simulink model "ElectricVehicleThermalManagementWithHeatPump"  (R2024b)
settings: Solver=VariableStepAuto  StartTime=0.0  StopTime=3600  RelTol=1e-3  AbsTol=1e-3
PreLoadFcn:
  | init_nmpc
InitFcn:
  | init_nmpc
model workspace: external: MATLAB File ElectricVehicleThermalManagementWithHeatPumpParameters.m (data not in the file)
values from neighbouring files (symbols this model uses):
  battery_C1_LUT = [1913.6 12447 30609 ... (first row only)    [ElectricVehicleThermalManagementWithHeatPumpParameters.m]
  battery_capacity_LUT = [280.081 276.25 276.392]    [ElectricVehicleThermalManagementWithHeatPumpParameters.m]
  battery_cell_cp = 795    [ElectricVehicleThermalManagementWithHeatPumpParameters.m]
  battery_cell_mass = 2.5    [ElectricVehicleThermalManagementWithHeatPumpParameters.m]
  battery_Em_LUT = [3.4966 3.5057 3.5148 ... (first row only)    [ElectricVehicleThermalManagementWithHeatPumpParameters.m]
  battery_N_cells = 20    [ElectricVehicleThermalManagementWithHeatPumpParameters.m]
  battery_Qe_init = 0    [ElectricVehicleThermalManagementWithHeatPumpParameters.m]
  battery_R0_LUT = [0.0117 0.0085 0.009 ... (first row only)    [ElectricVehicleThermalManagementWithHeatPumpParameters.m]
  battery_R1_LUT = [0.0109 0.0029 0.0013 ... (first row only)    [ElectricVehicleThermalManagementWithHeatPumpParameters.m]
  battery_SOC_LUT = [0; 0.1; 0.25; 0.5; 0.75; 0.9; 1]    [ElectricVehicleThermalManagementWithHeatPumpParameters.m]
  battery_T_init = -10    [ElectricVehicleThermalManagementWithHeatPumpParameters.m]
  battery_temperature_LUT = [5 20 40]    [ElectricVehicleThermalManagementWithHeatPumpParameters.m]
  cabin_duct_area = 0.04    [ElectricVehicleThermalManagementWithHeatPumpParameters.m]
  cabin_T_init = -10    [ElectricVehicleThermalManagementWithHeatPumpParameters.m]
  chiller_area_primary = 0.43982297150257105    (= 0.439822971503)    [ElectricVehicleThermalManagementWithHeatPumpParameters.m]
  chiller_N_baffles = 3    [ElectricVehicleThermalManagementWithHeatPumpParameters.m]
  chiller_N_tubes = 100    [ElectricVehicleThermalManagementWithHeatPumpParameters.m]
  chiller_tube_D = 0.0035    [ElectricVehicleThermalManagementWithHeatPumpParameters.m]
  chiller_tube_L = 0.4    [ElectricVehicleThermalManagementWithHeatPumpParameters.m]
  chiller_wall_conductivity = 240    [ElectricVehicleThermalManagementWithHeatPumpParameters.m]
  chiller_wall_thickness = 0.0001    [ElectricVehicleThermalManagementWithHeatPumpParameters.m]
  cond_evap_air_area_flow = 0.3906    [ElectricVehicleThermalManagementWithHeatPumpParameters.m]
  cond_evap_air_area_primary = 1.4834999999999998    (= 1.4835)    [ElectricVehicleThermalManagementWithHeatPumpParameters.m]
  cond_evap_W = 0.015    [ElectricVehicleThermalManagementWithHeatPumpParameters.m]
  cond_evap_wall_conductivity = 240    [ElectricVehicleThermalManagementWithHeatPumpParameters.m]
  cond_evap_wall_thickness = 0.0001    [ElectricVehicleThermalManagementWithHeatPumpParameters.m]
  coolant_channel_D = 0.0092    [ElectricVehicleThermalManagementWithHeatPumpParameters.m]
  coolant_pipe_D = 0.019    [ElectricVehicleThermalManagementWithHeatPumpParameters.m]
  coolant_T_init = -10    [ElectricVehicleThermalManagementWithHeatPumpParameters.m]
  coolant_tank_area = 0.0121    [ElectricVehicleThermalManagementWithHeatPumpParameters.m]
  coolant_tank_volume = 1.25    [ElectricVehicleThermalManagementWithHeatPumpParameters.m]
  coolant_valve_D_ratio_max = 0.95    [ElectricVehicleThermalManagementWithHeatPumpParameters.m]
  coolant_valve_D_ratio_min = 0.001    [ElectricVehicleThermalManagementWithHeatPumpParameters.m]
  coolant_valve_displacement = 0.0063    [ElectricVehicleThermalManagementWithHeatPumpParameters.m]
  coolant_valve_S_max = 0.0053    [ElectricVehicleThermalManagementWithHeatPumpParameters.m]
  evaporator_air_area_flow = 0.12    [ElectricVehicleThermalManagementWithHeatPumpParameters.m]
  evaporator_air_area_primary = 0.4323    [ElectricVehicleThermalManagementWithHeatPumpParameters.m]
  evaporator_W = 0.015    [ElectricVehicleThermalManagementWithHeatPumpParameters.m]
  evaporator_wall_conductivity = 240    [ElectricVehicleThermalManagementWithHeatPumpParameters.m]
  evaporator_wall_thickness = 0.0001    [ElectricVehicleThermalManagementWithHeatPumpParameters.m]
  expansion_valve_D_ratio_max = 0.9    [ElectricVehicleThermalManagementWithHeatPumpParameters.m]
  hex_area_primary = 0.070371675440411369    (= 0.0703716754404)    [ElectricVehicleThermalManagementWithHeatPumpParameters.m]
  hex_N_tubes = 64    [ElectricVehicleThermalManagementWithHeatPumpParameters.m]
  hex_tube_D = 0.0035    [ElectricVehicleThermalManagementWithHeatPumpParameters.m]
  hex_wall_conductivity = 240    [ElectricVehicleThermalManagementWithHeatPumpParameters.m]
  hex_wall_thickness = 0.0001    [ElectricVehicleThermalManagementWithHeatPumpParameters.m]
  inner_cond_air_area_flow = 0.1953    [ElectricVehicleThermalManagementWithHeatPumpParameters.m]
  inner_cond_air_area_primary = 0.99520000000000008    (= 0.9952)    [ElectricVehicleThermalManagementWithHeatPumpParameters.m]
  inner_cond_W = 0.02    [ElectricVehicleThermalManagementWithHeatPumpParameters.m]
  inner_cond_wall_conductivity = 240    [ElectricVehicleThermalManagementWithHeatPumpParameters.m]
  inner_cond_wall_thickness = 0.0001    [ElectricVehicleThermalManagementWithHeatPumpParameters.m]
  pump_speed_max = 1000    [ElectricVehicleThermalManagementWithHeatPumpParameters.m]
  radiator_air_area_flow = 0.097499999999999989    (= 0.0975)    [ElectricVehicleThermalManagementWithHeatPumpParameters.m]
  radiator_air_area_primary = 0.43687499999999996    (= 0.436875)    [ElectricVehicleThermalManagementWithHeatPumpParameters.m]
  radiator_W = 0.015    [ElectricVehicleThermalManagementWithHeatPumpParameters.m]
  radiator_wall_conductivity = 240    [ElectricVehicleThermalManagementWithHeatPumpParameters.m]
  radiator_wall_thickness = 0.0001    [ElectricVehicleThermalManagementWithHeatPumpParameters.m]
  refrigerant_p_init = 0.2    [ElectricVehicleThermalManagementWithHeatPumpParameters.m]
  refrigerant_pipe_D = 0.01    [ElectricVehicleThermalManagementWithHeatPumpParameters.m]
  refrigerant_valve_D_ratio_max = 0.95    [ElectricVehicleThermalManagementWithHeatPumpParameters.m]
  refrigerant_valve_displacement = 0.005    [ElectricVehicleThermalManagementWithHeatPumpParameters.m]
libraries: fl_lib x227, nesl_utility x162, SimscapeFluids_lib x30, LiBatteryElements_lib x16, slpidlib x3, SignalEditorBlockLib x1
(part 7 of 13)

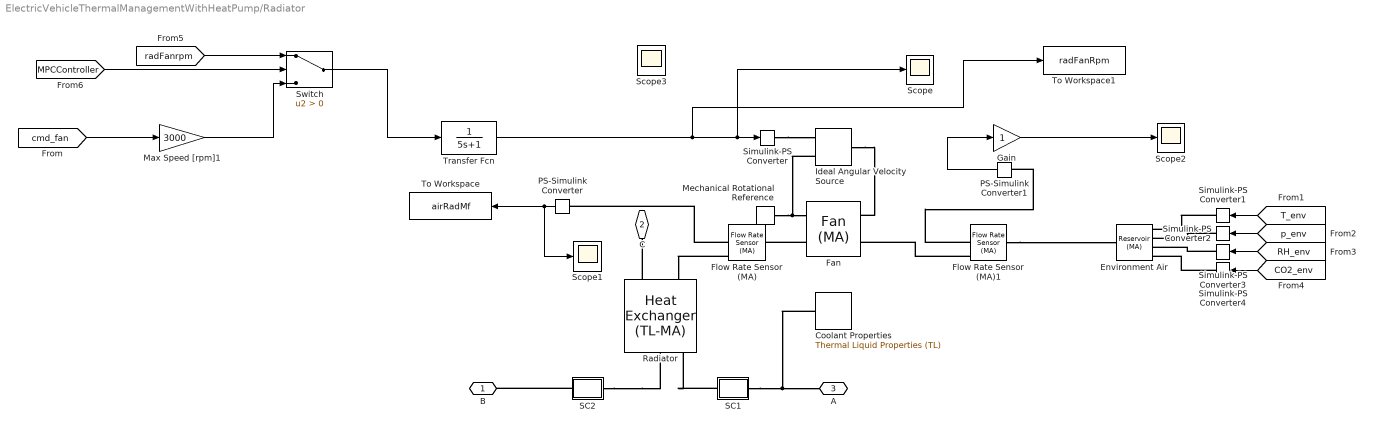
== system ElectricVehicleThermalManagementWithHeatPump/Radiator ==
  Coolant Properties : SimscapeFluids_lib/Thermal Liquid/Utilities/Thermal Liquid Properties (TL)  fluid_list=fluids.thermal_liquid.utilities.enum.thermal_liquid_fluid_list.ethylene_glycol  concentration_param_EG=fluids.thermal_liquid.utilities.enum.thermal_liquid_concentration.volume_fraction  concentration_param_PG=fluids.thermal_liquid.utilities.enum.thermal_liquid_concentration.volume_fraction  c_mass_SW=3.5e-3  c_mass_EG=0.1  c_mass_PG=0.1  c_mass_GL=0.1  c_vol_EG=0.5  c_vol_PG=0.1  beta_const_EG=2.1791 GPa  beta_const_PG=2.1791 GPa  beta_const_GL=2.1791 GPa  p_min_EG=0.01 MPa  p_min_PG=0.01 MPa  p_min_GL=0.01 MPa  p_max_EG=50 MPa  p_max_PG=50 MPa  p_max_GL=50 MPa  p_atm=0.101325 MPa  properties_range_check=simscape.enum.assert.action.error
  Environment Air : fl_lib/Moist Air/Elements/Reservoir (MA)  pressure_input=true  pressure_spec=foundation.enum.pressure_spec.atmospheric  reservoir_pressure=0.101325 MPa  temperature_input=true  temperature_spec=foundation.enum.temperature_spec.atmospheric  reservoir_temperature=293.15 K  humidity_input=true  humidity_spec=foundation.enum.HumiditySpec.RelativeHumidity  reservoir_RH=0.5  reservoir_x_w=0.01  reservoir_y_w=0.01  reservoir_HR=0.01  reservoir_Tw=287 K  trace_gas_input=true  trace_gas_spec=foundation.enum.trace_gas_spec.mole_fraction  reservoir_x_g=0.001  reservoir_y_g=0.001  water_droplets_input=false  reservoir_r_d=0  RH_ws=1  area_A=cabin_duct_area m^2  input_error_spec=foundation.enum.input_range_error.warn
      settings: InternalSimscapePortConfiguration="{\"Bottom\":[],\"Left\":[{\"id\":\"A\",\"label\":\"A\",\"type\":\"foundation.moist_air.moist_air\"}],\"Right\":[{\"id\":\"T\",\"label\":\"T\",\"type\":\"input\"},{\"id\":\"P\",\"label\":\"P\",\"type\":\"input\"},{\"id\":\"W\",\"label\":\"W\",\"type\":\"input\"},{\"id\":\"G\",\"label\":\"G\",\"type\":\"input\"}],\"Top\":[]}"
  Fan : SimscapeFluids_lib/Moist Air/Turbomachinery/Fan (MA)  fan_parameterization=fluids.moist_air.turbomachinery.enum.FanParameterization.Table1D  mechanical_power_spec=fluids.moist_air.turbomachinery.enum.FanMechanicalPowerSpec.Efficiency  flow_rate_nominal=0.8 m^3/s  pressure_nominal=400 Pa  eta_nominal=0.6  power_nominal=1620 W  pressure_max=600 Pa  flow_rate_max=1.5 m^3/s  omega_ref_nominal=1000 rpm  flow_rate_1D_TLU=[.0278, .0556, .0833, .111, .139, .167] m^3/s  pressure_1D_TLU=[6410, 6375, 6018, 5366, 4501, 3609] Pa  eta_1D_TLU=[.257, .394, .453, .47, .459, .415]  power_1D_TLU=[693, 900, 1107, 1267, 1363, 1452] W  omega_ref_1D=3000 rpm  rho_ref_1D=1.2 kg/m^3  omega_threshold_factor=1e-2  omega_dp_TLU=[2400; 3000; 3600] rpm  flow_rate_dp_TLU=[.0278, .0556, .0833, .111, .139, .167] m^3/s  pressure_dp_TLU=[4111, 4010, 3551, 2881, 2167, 1453; 6410, 6375, 6018, 5366, 4501, 3609; 9217, 9285, 9022, 8428, 7552, 6482] Pa  eta_dp_TLU=[.3, .434, .468, .459, .4, .3; .257, .394, .453, .47, .459, .415; .225, .359, .434, .461, .47, .459]  power_dp_TLU=[381, 514, 632, 697, 753, 809; 693, 900, 1107, 1267, 1363, 1452; 1139, 1438, 1732, 2029, 2233, 2358] W  rho_ref_dp=1.2 kg/m^3  omega_q_TLU=[2990; 3450; 3867] rpm  pressure_q_TLU=[31, 62, 93, 124] Pa  flow_rate_q_TLU=[.802, .759, .703, .611; .936, .902, .862, .81; 1.056, 1.027, .994, .956] m^3/s  eta_q_TLU=[.088, .162, .22, .261; .068, .128, .18, .222; .055, .105, .148, .188]  power_q_TLU=[283, 290, 297, 290; 427, 437, 445, 452; 595, 606, 625, 631] W  rho_ref_q=1.2 kg/m^3  diameter_ratio=1  mech_orientation=fluids.moist_air.turbomachinery.enum.FanMechanicalOrientation.Positive  area_A=cabin_duct_area m^2  area_B=cabin_duct_area m^2
      settings: InternalSimscapePortConfiguration="{\"Bottom\":[],\"Left\":[{\"id\":\"A\",\"label\":\"A\",\"type\":\"foundation.moist_air.moist_air\"},{\"id\":\"C\",\"label\":\"C\",\"type\":\"foundation.mechanical.rotational.rotational\"}],\"Right\":[{\"id\":\"B\",\"label\":\"B\",\"type\":\"foundation.moist_air.moist_air\"},{\"id\":\"R\",\"label\":\"R\",\"type\":\"foundation.mechanical.rotational.rotational\"}],\"Top\":[]}"
  Flow Rate Sensor (MA) : fl_lib/Moist Air/Sensors/Flow Rate Sensor (MA)  mass_flow_measure=true  volumetric_flow_measure=false  volumetric_flow_conditions=foundation.enum.volumetric_flow_conditions.actual  p_std=0.101325 MPa  T_std=20 degC  RH_std=0.65  energy_flow_measure=true  vapor_flow_measure=false  gas_flow_measure=false  droplets_flow_measure=false
      settings: InternalSimscapePortConfiguration="{\"Bottom\":[{\"id\":\"PHI\",\"label\":\"φ\",\"type\":\"output\"}],\"Left\":[{\"id\":\"A\",\"label\":\"A\",\"type\":\"foundation.moist_air.moist_air\"}],\"Right\":[{\"id\":\"B\",\"label\":\"B\",\"type\":\"foundation.moist_air.moist_air\"},{\"id\":\"M\",\"label\":\"M\",\"type\":\"output\"}],\"Top\":[]}"
  Flow Rate Sensor (MA)1 : fl_lib/Moist Air/Sensors/Flow Rate Sensor (MA)  mass_flow_measure=true  volumetric_flow_measure=false  volumetric_flow_conditions=foundation.enum.volumetric_flow_conditions.actual  p_std=0.101325 MPa  T_std=20 degC  RH_std=0.65  energy_flow_measure=true  vapor_flow_measure=false  gas_flow_measure=false  droplets_flow_measure=false
      settings: InternalSimscapePortConfiguration="{\"Bottom\":[{\"id\":\"PHI\",\"label\":\"φ\",\"type\":\"output\"}],\"Left\":[{\"id\":\"A\",\"label\":\"A\",\"type\":\"foundation.moist_air.moist_air\"}],\"Right\":[{\"id\":\"B\",\"label\":\"B\",\"type\":\"foundation.moist_air.moist_air\"},{\"id\":\"M\",\"label\":\"M\",\"type\":\"output\"}],\"Top\":[]}"
  Gain : Gain
  Ideal Angular Velocity Source : fl_lib/Mechanical/Mechanical Sources/Ideal Angular Velocity Source
  Max Speed [rpm]1 : Gain  Gain=3000
  Mechanical Rotational Reference : fl_lib/Mechanical/Rotational Elements/Mechanical Rotational Reference
  PS-Simulink Converter : nesl_utility/PS-Simulink Converter  PhysicalDomain=network_engine_domain  SubClassName=ps_output  LeftPortType=input  RightPortType=output  PseudoPeriodic=off  Frequencies=[]  VectorFormat=inherit  Unit=inherit  AffineConversion=off
  PS-Simulink Converter1 : nesl_utility/PS-Simulink Converter  PhysicalDomain=network_engine_domain  SubClassName=ps_output  LeftPortType=input  RightPortType=output  PseudoPeriodic=off  Frequencies=[]  VectorFormat=inherit  Unit=inherit  AffineConversion=off
  Radiator : SimscapeFluids_lib/Heat Exchangers/Thermal Liquid - Moist Air/Heat Exchanger (TL-MA)  flow_arrangement=fluids.heat_exchangers.enum.FlowArrangementTLMA.Cross  cross_flow_arrangement=fluids.heat_exchangers.enum.CrossFlowArrangementTLMA.MixedUnmixed  R_wall=radiator_wall_thickness / radiator_air_area_primary / radiator_wall_conductivity K/W  area_A1=pi * coolant_pipe_D^2 / 4 m^2  area_B1=pi * coolant_pipe_D^2 / 4 m^2  area_A2=cabin_duct_area m^2  area_B2=cabin_duct_area m^2  flow_geometry_TL=fluids.heat_exchangers.enum.FlowGeometryTL.InsideTubes  tube_num_TL=radiator_N_tubes  tube_length_TL=radiator_L m  tube_cross_section_TL=fluids.heat_exchangers.enum.TubeCrossSection.Rectangular  tube_diameter_TL=0.1 m  tube_width_TL=radiator_W m  tube_height_TL=radiator_tube_H m  tube_inner_diameter_TL=0.05 m  tube_outer_diameter_TL=0.1 m  tube_flow_area_TL=0.01 m^2  tube_wetted_perimeter_TL=0.4 m  tube_heat_perimeter_TL=0.4 m  tube_pressure_loss_spec_TL=fluids.heat_exchangers.enum.TubePressureLossSpec.Haaland  tube_loss_coeff_TL=10  tube_local_pressure_loss_spec_TL=fluids.heat_exchangers.enum.LocalLossSpec.AggregateLength  tube_length_add_TL=radiator_tube_Leq m  tube_local_loss_coefficient_TL=0.1  tube_roughness_pressure_TL=15e-6 m  tube_Re_lam_pressure_TL=2000  tube_Re_tur_pressure_TL=4000  tube_shape_factor_generic_TL=64  tube_heat_coeff_spec_TL=fluids.heat_exchangers.enum.TubeHeatCoeffSpec.Gneilinski  tube_colburn_coeff_TL=[.023, .8, .33]  tube_roughness_heat_TL=15e-6 m  tube_Re_lam_heat_TL=2000  tube_Re_tur_heat_TL=4000  tube_Nu_lam_generic_TL=3.66  bank_arrangement_TL=fluids.heat_exchangers.enum.BankArrangement.Inline  bank_num_rows_TL=5  bank_tubes_per_row_TL=5  bank_width_TL=1 m  bank_tube_diameter_TL=0.05 m  bank_longitudinal_pitch_TL=0.15 m  bank_transverse_pitch_TL=0.15 m  bank_pressure_loss_spec_TL=fluids.heat_exchangers.enum.BankPressureLossSpec.Martin  bank_euler_TL=10  bank_heat_coeff_spec_TL=fluids.heat_exchangers.enum.BankHeatCoeffSpec.Martin  bank_colburn_coeff_TL=[.27, .63, .36]  generic_flow_area_TL=0.01 m^2  generic_heat_area_TL=2 m^2  generic_volume_TL=0.05 m^3  generic_loss_coeff_TL=10  generic_colburn_coeff_TL=[.023, .8, .33]  fouling_factor_TL=0.1 m^2*K/kW  fin_area_TL=0 m^2  fin_efficiency_TL=0  p_init_TL=coolant_p_init MPa  T_init_TL=coolant_T_init degC  flow_geometry_MA=fluids.heat_exchangers.enum.FlowGeometryMA.Generic  tube_num_MA=1  tube_length_MA=5 m  tube_cross_section_MA=fluids.heat_exchangers.enum.TubeCrossSection.Circular  tube_diameter_MA=0.1 m  tube_width_MA=0.1 m  tube_height_MA=0.1 m  tube_inner_diameter_MA=0.05 m  tube_outer_diameter_MA=0.1 m  tube_flow_area_MA=0.01 m^2  tube_wetted_perimeter_MA=0.4 m  tube_heat_perimeter_MA=0.4 m  tube_pressure_loss_spec_MA=fluids.heat_exchangers.enum.TubePressureLossSpec.Haaland  tube_loss_coeff_MA=10  tube_local_pressure_loss_spec_MA=fluids.heat_exchangers.enum.LocalLossSpec.AggregateLength  tube_length_add_MA=0.1 m  tube_local_loss_coefficient_MA=0.1  tube_roughness_pressure_MA=15e-6 m  tube_Re_lam_pressure_MA=2000  tube_Re_tur_pressure_MA=4000  tube_shape_factor_generic_MA=64  tube_heat_coeff_spec_MA=fluids.heat_exchangers.enum.TubeHeatCoeffSpec.Gneilinski  tube_colburn_coeff_MA=[.023, .8, .33]  tube_roughness_heat_MA=15e-6 m  tube_Re_lam_heat_MA=2000  tube_Re_tur_heat_MA=4000  tube_Nu_lam_generic_MA=3.66  bank_arrangement_MA=fluids.heat_exchangers.enum.BankArrangement.Inline  bank_num_rows_MA=5  bank_tubes_per_row_MA=5  bank_width_MA=1 m  bank_tube_diameter_MA=0.05 m  bank_longitudinal_pitch_MA=0.15 m  bank_transverse_pitch_MA=0.15 m  bank_pressure_loss_spec_MA=fluids.heat_exchangers.enum.BankPressureLossSpec.Martin  bank_euler_MA=10  bank_heat_coeff_spec_MA=fluids.heat_exchangers.enum.BankHeatCoeffSpec.Martin  bank_colburn_coeff_MA=[.27, .63, .36]  generic_flow_area_MA=radiator_air_area_flow m^2  generic_heat_area_MA=radiator_air_area_primary m^2  generic_volume_MA=radiator_air_area_flow * radiator_W m^3  generic_loss_coeff_MA=10  generic_colburn_coeff_MA=[0.27, 0.63, 0.36]  fouling_factor_MA=0.1 m^2*K/kW  fin_area_MA=radiator_air_area_fins m^2  fin_efficiency_MA=0.7  p_init_MA=cabin_p_init MPa  T_init_MA=cabin_T_init degC  humidity_spec_MA=foundation.enum.HumiditySpec.RelativeHumidity  RH_init_MA=cabin_RH_init  x_w_init_MA=0.01  y_w_init_MA=0.01  HR_init_MA=0.01  Tw_init_MA=287 K  trace_gas_spec_MA=foundation.enum.trace_gas_spec.mole_fraction  x_g_init_MA=0.001  y_g_init_MA=cabin_CO2_init  r_d_init_MA=0  RH_ws_MA=1  time_constant_cond_MA=1e-3 s  time_constant_evap_MA=1e-3 s  fraction_entrained_MA=1
      settings: InternalSimscapePortConfiguration="{\"Bottom\":[],\"Left\":[{\"id\":\"A1\",\"label\":\"A1\",\"type\":\"foundation.thermal_liquid.thermal_liquid\"},{\"id\":\"B1\",\"label\":\"B1\",\"type\":\"foundation.thermal_liquid.thermal_liquid\"}],\"Right\":[{\"id\":\"A2\",\"label\":\"A2\",\"type\":\"foundation.moist_air.moist_air\"},{\"id\":\"B2\",\"label\":\"B2\",\"type\":\"foundation.moist_air.moist_air\"}],\"Top\":[{\"id\":\"W\",\"label\":\"W\",\"type\":\"output\"}]}"
  SC1 : Subsystem
  SC2 : Subsystem
  Scope{,1..3} (4 alike) : Scope
  Simulink-PS Converter : nesl_utility/Simulink-PS Converter  PhysicalDomain=network_engine_domain  SubClassName=ps_input  LeftPortType=input  RightPortType=output  PseudoPeriodic=off  Frequencies=[]  NoiseDistribution=none  NoiseParameters=[]  Unit=rpm  AffineConversion=off  FilteringAndDerivatives=provide  SimscapeFilterOrder=1  InputFilterTimeConstant=0.001  UdotUserProvided=0
  Simulink-PS Converter1 : nesl_utility/Simulink-PS Converter  PhysicalDomain=network_engine_domain  SubClassName=ps_input  LeftPortType=input  RightPortType=output  PseudoPeriodic=off  Frequencies=[]  NoiseDistribution=none  NoiseParameters=[]  Unit=degC  AffineConversion=on  FilteringAndDerivatives=provide  SimscapeFilterOrder=1  InputFilterTimeConstant=0.001  UdotUserProvided=0
  Simulink-PS Converter2 : nesl_utility/Simulink-PS Converter  PhysicalDomain=network_engine_domain  SubClassName=ps_input  LeftPortType=input  RightPortType=output  PseudoPeriodic=off  Frequencies=[]  NoiseDistribution=none  NoiseParameters=[]  Unit=MPa  AffineConversion=off  FilteringAndDerivatives=provide  SimscapeFilterOrder=1  InputFilterTimeConstant=0.001  UdotUserProvided=0
  Simulink-PS Converter3 : nesl_utility/Simulink-PS Converter  PhysicalDomain=network_engine_domain  SubClassName=ps_input  LeftPortType=input  RightPortType=output  PseudoPeriodic=off  Frequencies=[]  NoiseDistribution=none  NoiseParameters=[]  Unit=1  AffineConversion=off  FilteringAndDerivatives=provide  SimscapeFilterOrder=1  InputFilterTimeConstant=0.001  UdotUserProvided=0
  Simulink-PS Converter4 : nesl_utility/Simulink-PS Converter  PhysicalDomain=network_engine_domain  SubClassName=ps_input  LeftPortType=input  RightPortType=output  PseudoPeriodic=off  Frequencies=[]  NoiseDistribution=none  NoiseParameters=[]  Unit=1  AffineConversion=off  FilteringAndDerivatives=provide  SimscapeFilterOrder=1  InputFilterTimeConstant=0.001  UdotUserProvided=0
  Switch : Switch  Criteria=u2 > Threshold  SaturateOnIntegerOverflow=off  InputSameDT=off
  To Workspace : ToWorkspace  VariableName=airRadMf  SampleTime=-1
  To Workspace1 : ToWorkspace  VariableName=radFanRpm  SampleTime=-1
  Transfer Fcn : TransferFcn  Denominator=[5 1]
  B : PMIOPort  Side=Left
  C : PMIOPort  Port=2  Side=Left
  A : PMIOPort  Port=3  Side=Right
  wires:
  [T_env] -> Simulink-PS Converter1/1
  [p_env] -> Simulink-PS Converter2/1
  [RH_env] -> Simulink-PS Converter3/1
  [CO2_env] -> Simulink-PS Converter4/1
  PS-Simulink Converter/1 -> Scope1/1, To Workspace/1
  PS-Simulink Converter1/1 -> Gain/1
  Gain/1 -> Scope2/1
  Transfer Fcn/1 -> To Workspace1/1, Scope/1, Simulink-PS Converter/1
  [radFanrpm] -> Switch/1
  [cmd_fan] -> Max Speed [rpm]1/1
  Switch/1 -> Transfer Fcn/1
  Max Speed [rpm]1/1 -> Switch/3
  [MPCController] -> Switch/2
  connections:
  SC2/LConn1 -- Radiator/LConn2
  SC1/RConn1 -- Radiator/LConn1
  Radiator/RConn2 -- C/RConn1
  Simulink-PS Converter2/RConn1 -- Environment Air/RConn2
  Simulink-PS Converter4/RConn1 -- Environment Air/RConn4
  Simulink-PS Converter3/RConn1 -- Environment Air/RConn3
  Simulink-PS Converter1/RConn1 -- Environment Air/RConn1
  SC2/RConn1 -- B/RConn1
  SC1/LConn1 -- Coolant Properties/RConn1 -- A/RConn1
  Ideal Angular Velocity Source/RConn2 -- Mechanical Rotational Reference/LConn1 -- Fan/LConn2
  Simulink-PS Converter/RConn1 -- Ideal Angular Velocity Source/RConn1
  Ideal Angular Velocity Source/LConn1 -- Fan/RConn2
  Fan/LConn1 -- Flow Rate Sensor (MA)/LConn1
  Flow Rate Sensor (MA)/RConn1 -- Radiator/RConn1
  Flow Rate Sensor (MA)/RConn2 -- PS-Simulink Converter/LConn1
  Flow Rate Sensor (MA)1/LConn1 -- Environment Air/LConn1
  Flow Rate Sensor (MA)1/RConn1 -- Fan/RConn1
  Flow Rate Sensor (MA)1/RConn2 -- PS-Simulink Converter1/LConn1

== system ElectricVehicleThermalManagementWithHeatPump/Radiator Bypass Valve ==
  Bias : Bias  Bias=-1  SaturateOnIntegerOverflow=off
  Gain : Gain  Gain=2
  Max Valve Displacement [m] : Gain  Gain=coolant_valve_displacement
  Radiator Bypass Valve : SimscapeFluids_lib/Thermal Liquid/Valves & Orifices/Directional Control Valves/3-Way Directional Valve (TL)  open_orifices_pos=fluids.thermal_liquid.valves.directional_control_valves.enum.OpenOrifices3Way.PA  open_orifices_neg=fluids.thermal_liquid.valves.directional_control_valves.enum.OpenOrifices3Way.AT  area_spec=fluids.thermal_liquid.valves.directional_control_valves.enum.area_spec.identical  valve_spec=fluids.thermal_liquid.valves.enum.orifice_spec.linear  del_S_max=coolant_valve_displacement m  area_max=pi * (coolant_valve_D_ratio_max*coolant_pipe_D)^2 / 4 m^2  del_S_TLU=[0 0.002 0.004 0.007 0.017] m  valve_area_TLU=[1e-09, 2.0352e-07, 4.0736e-05, .00011438, .00034356] m^2  del_S_flow_TLU=[0 0.002 0.004 0.007 0.017] m  p_diff_TLU=[-.1, .3, .5, .7] MPa  vol_flow_TLU=1e-3 * [1.7e-05, 2e-05, 2.6e-05; .0035, .0045, .0053; .7, .9, 1.06; 1.96, 2.5, 3; 6, 7.7, 9.13] m^3/s  mdot_TLU=[-1e-05, 1.7e-05, 2e-05, 2.6e-05; -.002, .0035, .0045, .0053; -.4, .7, .9, 1.06; -1.13, 1.96, 2.5, 3; -3.45, 6, 7.7, 9.13] kg/s  T_ref_in=293.15 K  p_ref_in=0.101325 MPa  area_leak=pi * (coolant_valve_D_ratio_min*coolant_pipe_D)^2 / 4 m^2  Cd=0.7  Re_c=150  smoothing_factor=0.01  pressure_recovery=simscape.enum.onoff.on  area=pi * coolant_pipe_D^2 / 4 m^2  S_max_PA=coolant_valve_S_max m  del_S_max_PA=coolant_valve_displacement-(coolant_valve_displacement)*(pi * (coolant_valve_D_ratio_min*coolant_pipe_D)^2 / 4)/(pi * (coolant_valve_D_ratio_max*coolant_pipe_D)^2 / 4) m  area_max_PA=pi * (coolant_valve_D_ratio_max*coolant_pipe_D)^2 / 4 m^2  del_S_TLU_PA=[0 0.002 0.004 0.007 0.017] m  valve_area_TLU_PA=[1e-09, 2.0352e-07, 4.0736e-05, .00011438, .00034356] m^2  del_S_flow_TLU_PA=[0 0.002 0.004 0.007 0.017] m  p_diff_TLU_PA=[-.1, .3, .5, .7] MPa  vol_flow_TLU_PA=1e-3 * [1.7e-05, 2e-05, 2.6e-05; .0035, .0045, .0053; .7, .9, 1.06; 1.96, 2.5, 3; 6, 7.7, 9.13] m^3/s  mdot_TLU_PA=[-1e-05, 1.7e-05, 2e-05, 2.6e-05; -.002, .0035, .0045, .0053; -.4, .7, .9, 1.06; -1.13, 1.96, 2.5, 3; -3.45, 6, 7.7, 9.13] kg/s  S_max_AT=-coolant_valve_S_max m  del_S_max_AT=coolant_valve_displacement-(coolant_valve_displacement)*(pi * (coolant_valve_D_ratio_min*coolant_pipe_D)^2 / 4)/(pi * (coolant_valve_D_ratio_max*coolant_pipe_D)^2 / 4) m  area_max_AT=pi * (coolant_valve_D_ratio_max*coolant_pipe_D)^2 / 4 m^2  del_S_TLU_AT=[0 0.002 0.004 0.007 0.017] m  valve_area_TLU_AT=[1e-09, 2.0352e-07, 4.0736e-05, .00011438, .00034356] m^2  del_S_flow_TLU_AT=[0 0.002 0.004 0.007 0.017] m  p_diff_TLU_AT=[-.1, .3, .5, .7] MPa  vol_flow_TLU_AT=1e-3 * [1.7e-05, 2e-05, 2.6e-05; .0035, .0045, .0053; .7, .9, 1.06; 1.96, 2.5, 3; 6, 7.7, 9.13] m^3/s  mdot_TLU_AT=[-1e-05, 1.7e-05, 2e-05, 2.6e-05; -.002, .0035, .0045, .0053; -.4, .7, .9, 1.06; -1.13, 1.96, 2.5, 3; -3.45, 6, 7.7, 9.13] kg/s  S_max_PT=2.5e-3 m  del_S_max_PT=0.005 m  area_max_PT=1e-4 m^2  del_S_TLU_PT=[0, .002, .004, .007, .017] m  valve_area_TLU_PT=[1e-09, 2.0352e-07, 4.0736e-05, .00011438, .00034356] m^2  del_S_flow_TLU_PT=[0, .002, .004, .007, .017] m  p_diff_TLU_PT=[.3, .5, .7] MPa  vol_flow_TLU_PT=1e-3 * [1.7e-05, 2e-05, 2.6e-05; .0035, .0045, .0053; .7, .9, 1.06; 1.96, 2.5, 3; 6, 7.7, 9.13] m^3/s  mdot_TLU_PT=[1.7e-05, 2e-05, 2.6e-05; .0035, .0045, .0053; .7, .9, 1.06; 1.96, 2.5, 3; 6, 7.7, 9.13] kg/s
      settings: InternalSimscapePortConfiguration="{\"Bottom\":[],\"Left\":[{\"id\":\"A\",\"label\":\"A\",\"type\":\"foundation.thermal_liquid.thermal_liquid\"}],\"Right\":[{\"id\":\"S\",\"label\":\"S\",\"type\":\"input\"},{\"id\":\"P\",\"label\":\"P\",\"type\":\"foundation.thermal_liquid.thermal_liquid\"},{\"id\":\"T\",\"label\":\"T\",\"type\":\"foundation.thermal_liquid.thermal_liquid\"}],\"Top\":[]}"
  Scope : Scope
  Simulink-PS Converter : nesl_utility/Simulink-PS Converter  PhysicalDomain=network_engine_domain  SubClassName=ps_input  LeftPortType=input  RightPortType=output  PseudoPeriodic=off  Frequencies=[]  NoiseDistribution=none  NoiseParameters=[]  Unit=m  AffineConversion=off  FilteringAndDerivatives=provide  SimscapeFilterOrder=1  InputFilterTimeConstant=0.001  UdotUserProvided=0
  Transfer Fcn : TransferFcn  Denominator=[1 1]
  B : PMIOPort  Side=Left
  C : PMIOPort  Port=2  Side=Left
  A : PMIOPort  Port=3  Side=Right
  wires:
  Gain/1 -> Bias/1
  [cmd_rad_bypass] -> Scope/1, Transfer Fcn/1
  Bias/1 -> Max Valve Displacement [m]/1
  Transfer Fcn/1 -> Gain/1
  Max Valve Displacement [m]/1 -> Simulink-PS Converter/1
  connections:
  Radiator Bypass Valve/LConn1 -- A/RConn1
  B/RConn1 -- Radiator Bypass Valve/RConn2
  Radiator Bypass Valve/RConn1 -- Simulink-PS Converter/RConn1
  Radiator Bypass Valve/RConn3 -- C/RConn1

== system ElectricVehicleThermalManagementWithHeatPump/Scenario ==
  note: Environment
  note: Cabin HVAC
  CO2 Fraction : Constant  Value=4e-4
  Clock : Clock
  Desired Temperature [degC] : Constant  Value=21
  Number of Occupants : Constant
  Power Demand : Subsystem
  Pressure [MPa] : Constant  Value=0.101325
  Relative Humidity : Constant  Value=0.5
  Scope : Scope
  Scope1 : Scope
  Scope2 : Scope
  Temperature [degC] : Constant  Value=-10
  Temperature [degC] vs Time : Lookup_n-D  NumberOfTableDimensions=1  BreakpointsForDimension1=[0 1150 1800 3600]  Table=[25 25 5 5]  InternalRulePriority=Speed  RndMeth=Simplest
  To Workspace : ToWorkspace  VariableName=batA_meas  SampleTime=-1
  Variant Source : VariantSource  VariantControlMode=label  LabelModeActiveChoice=constant
      settings: AttributesFormatString=%<LabelModeActiveChoice>
  Vehicle Speed [km/hr] : SignalEditorBlockLib/Signal Editor  FileName=ElectricVehicleThermalManagementWithHeatPumpVehicleSpeed.mat  ActiveScenario=DriveCycle  ActiveSignal=speed  IsBus=off  OutputBusObjectStr=Bus: BusObject  SampleTime=0  ZeroCross=off  OutputAfterFinalValue=Extrapolation  Unit=inherit  PreserveSignalName=on  ApplySigPropsToAllScenarios=on  ApplySigPropsToAllSignals=off
  tag scope: CO2_env=global, I_battery=global, N_occupant=global, Q_charger=global, Q_dcdc=global, Q_inverter=global, Q_motor=global, RH_env=global, T_desired=global, T_env=global, p_env=global, v_vehicle=global
  wires:
  Vehicle Speed [km/hr]/1 -> [v_vehicle], Power Demand/1(speed)
  Pressure [MPa]/1 -> [p_env]
  CO2 Fraction/1 -> [CO2_env]
  Desired Temperature [degC]/1 -> [T_desired]
  Relative Humidity/1 -> [RH_env]
  Power Demand/1(I_battery) -> To Workspace/1, Scope1/1, [I_battery]
  Power Demand/2(Q_inverter) -> [Q_inverter]
  Power Demand/3(Q_motor) -> Scope2/1, [Q_motor]
  Power Demand/4(Q_charger) -> [Q_charger]
  Power Demand/5(Q_dcdc) -> Scope/1, [Q_dcdc]
  Number of Occupants/1 -> [N_occupant]
  Variant Source/1 -> [T_env]
  Temperature [degC]/1 -> Variant Source/1
  Clock/1 -> Temperature [degC] vs Time/1
  Temperature [degC] vs Time/1 -> Variant Source/2

== system ElectricVehicleThermalManagementWithHeatPump/Battery/Pack 1 ==
  note: Scale up voltage drop
      | to total of N cells
  Controlled Voltage Source : fl_lib/Electrical/Electrical Sources/Controlled Voltage Source
  Lithium Cell 1RC : Subsystem
      settings: PortSchema="{\"entries\":[{\"content\":{\"sides\":[{\"content\":{\"connectorIds\":[]},\"type\":\"ConnectorPlacement.EquallySpacedRectSide\",\"uuid\":\"ccb9f794-c2a7-49a2-9836-26607ca18a9f\"},{\"content\":{\"connectorIds\":[],\"side\":\"RIGHT\"},\"type\":\"ConnectorPlacement.EquallySpacedRectSide\",\"uuid\":\"f1620ab9-2b03-42d4-871e-d35b8093f316\"},{\"content\":{\"connectorIds\":[\"LConn1\",\"LConn2\"],\"side\":\"TOP\"},\"type\":\"ConnectorPlacement.EquallySpacedRectSide\",\"uuid\":\"e679b0d8-ccbe-4539-8d6b-f3ffcd05b92b\"},{\"content\":{\"connectorIds\":[\"RConn1\",\"RConn2\"],\"side\":\"BOTTOM\"},\"type\":\"ConnectorPlacement.EquallySpacedRectSide\",\"uuid\":\"2833ed9d-c0e8-49c1-ad7b-8d4bc87d1df9\"},{\"content\":{\"connectorIds\":[],\"side\":\"HIDDEN\"},\"type\":\"ConnectorPlacement.EquallySpacedRectSide\",\"uuid\":\"76338804-e613-4140-a6be-ae9642a12407\"}]},\"type\":\"ConnectorPlacement.EquallySpacedConnector\",\"uuid\":\"276130fc-4c62-4f99-ae12-f3121ff878f4\"}],\"packageUris\":[\"http://schema.mathworks.com/mf0/Connector/R2020b\"],\"version\":\"1.0\"}"
      mask Display:
      | % Battery icon
      | plot([0 0 0.8 0.8], [0.2 0.9 0.9 1.5])
      | plot([0 0 0.8 0.8], -[0.2 0.9 0.9 1.5])
      | patch([-0.4 0.4 0.4 -0.4], [-0.45 -0.45 -0.15 -0.15], [0 0 0])
      | patch([-0.9 0.9 0.9 -0.9], [0.15 0.15 0.45 0.45], [0 0 0])
      | 
      | % Plot points to set plot range
      | color('white')
      | plot(1.5,1.5)
      | plot(-1.5,-1.5)
      | 
      | % Port labels
      | color('red')
      | port_label('LConn',1,'P')
      | port_label('LConn',2,'+')
      | port_label('RConn',1,'T')
      | port_label('RConn',2,'-')
  N : fl_lib/Physical Signals/Functions/PS Gain  gain=Ncells
  N-1 : fl_lib/Physical Signals/Functions/PS Gain  gain=Ncells - 1
  Thermal Model : Subsystem
  Voltage Sensor : fl_lib/Electrical/Electrical Sensors/Voltage Sensor
  - : PMIOPort  Side=Right
  H : PMIOPort  Port=2  Side=Left
  + : PMIOPort  Port=3  Side=Left
  connections:
  N/RConn1 -- Thermal Model/LConn2
  H/RConn1 -- Thermal Model/LConn1
  -/RConn1 -- Controlled Voltage Source/RConn2
  N-1/RConn1 -- Controlled Voltage Source/RConn1
  +/RConn1 -- Lithium Cell 1RC/LConn2 -- Voltage Sensor/LConn1
  Voltage Sensor/RConn1 -- N-1/LConn1
  Lithium Cell 1RC/RConn2 -- Voltage Sensor/RConn2 -- Controlled Voltage Source/LConn1
  Lithium Cell 1RC/RConn1 -- Thermal Model/RConn1
  Lithium Cell 1RC/LConn1 -- N/LConn1

== system ElectricVehicleThermalManagementWithHeatPump/Battery/Pack 2 ==
  note: Scale up voltage drop
      | to total of N cells
  Controlled Voltage Source : fl_lib/Electrical/Electrical Sources/Controlled Voltage Source
  Lithium Cell 1RC : Subsystem
      settings: PortSchema="{\"entries\":[{\"content\":{\"sides\":[{\"content\":{\"connectorIds\":[]},\"type\":\"ConnectorPlacement.EquallySpacedRectSide\",\"uuid\":\"ccb9f794-c2a7-49a2-9836-26607ca18a9f\"},{\"content\":{\"connectorIds\":[],\"side\":\"RIGHT\"},\"type\":\"ConnectorPlacement.EquallySpacedRectSide\",\"uuid\":\"f1620ab9-2b03-42d4-871e-d35b8093f316\"},{\"content\":{\"connectorIds\":[\"LConn1\",\"LConn2\"],\"side\":\"TOP\"},\"type\":\"ConnectorPlacement.EquallySpacedRectSide\",\"uuid\":\"e679b0d8-ccbe-4539-8d6b-f3ffcd05b92b\"},{\"content\":{\"connectorIds\":[\"RConn1\",\"RConn2\"],\"side\":\"BOTTOM\"},\"type\":\"ConnectorPlacement.EquallySpacedRectSide\",\"uuid\":\"2833ed9d-c0e8-49c1-ad7b-8d4bc87d1df9\"},{\"content\":{\"connectorIds\":[],\"side\":\"HIDDEN\"},\"type\":\"ConnectorPlacement.EquallySpacedRectSide\",\"uuid\":\"76338804-e613-4140-a6be-ae9642a12407\"}]},\"type\":\"ConnectorPlacement.EquallySpacedConnector\",\"uuid\":\"276130fc-4c62-4f99-ae12-f3121ff878f4\"}],\"packageUris\":[\"http://schema.mathworks.com/mf0/Connector/R2020b\"],\"version\":\"1.0\"}"
      mask Display:
      | % Battery icon
      | plot([0 0 0.8 0.8], [0.2 0.9 0.9 1.5])
      | plot([0 0 0.8 0.8], -[0.2 0.9 0.9 1.5])
      | patch([-0.4 0.4 0.4 -0.4], [-0.45 -0.45 -0.15 -0.15], [0 0 0])
      | patch([-0.9 0.9 0.9 -0.9], [0.15 0.15 0.45 0.45], [0 0 0])
      | 
      | % Plot points to set plot range
      | color('white')
      | plot(1.5,1.5)
      | plot(-1.5,-1.5)
      | 
      | % Port labels
      | color('red')
      | port_label('LConn',1,'P')
      | port_label('LConn',2,'+')
      | port_label('RConn',1,'T')
      | port_label('RConn',2,'-')
  N : fl_lib/Physical Signals/Functions/PS Gain  gain=Ncells
  N-1 : fl_lib/Physical Signals/Functions/PS Gain  gain=Ncells - 1
  Thermal Model : Subsystem
  Voltage Sensor : fl_lib/Electrical/Electrical Sensors/Voltage Sensor
  - : PMIOPort  Side=Right
  H : PMIOPort  Port=2  Side=Left
  + : PMIOPort  Port=3  Side=Left
  connections:
  N/RConn1 -- Thermal Model/LConn2
  H/RConn1 -- Thermal Model/LConn1
  -/RConn1 -- Controlled Voltage Source/RConn2
  N-1/RConn1 -- Controlled Voltage Source/RConn1
  +/RConn1 -- Lithium Cell 1RC/LConn2 -- Voltage Sensor/LConn1
  Voltage Sensor/RConn1 -- N-1/LConn1
  Lithium Cell 1RC/RConn2 -- Voltage Sensor/RConn2 -- Controlled Voltage Source/LConn1
  Lithium Cell 1RC/RConn1 -- Thermal Model/RConn1
  Lithium Cell 1RC/LConn1 -- N/LConn1

== system ElectricVehicleThermalManagementWithHeatPump/Battery/Pack 3 ==
  note: Scale up voltage drop
      | to total of N cells
  Controlled Voltage Source : fl_lib/Electrical/Electrical Sources/Controlled Voltage Source
  Lithium Cell 1RC : Subsystem
      settings: PortSchema="{\"entries\":[{\"content\":{\"sides\":[{\"content\":{\"connectorIds\":[]},\"type\":\"ConnectorPlacement.EquallySpacedRectSide\",\"uuid\":\"ccb9f794-c2a7-49a2-9836-26607ca18a9f\"},{\"content\":{\"connectorIds\":[],\"side\":\"RIGHT\"},\"type\":\"ConnectorPlacement.EquallySpacedRectSide\",\"uuid\":\"f1620ab9-2b03-42d4-871e-d35b8093f316\"},{\"content\":{\"connectorIds\":[\"LConn1\",\"LConn2\"],\"side\":\"TOP\"},\"type\":\"ConnectorPlacement.EquallySpacedRectSide\",\"uuid\":\"e679b0d8-ccbe-4539-8d6b-f3ffcd05b92b\"},{\"content\":{\"connectorIds\":[\"RConn1\",\"RConn2\"],\"side\":\"BOTTOM\"},\"type\":\"ConnectorPlacement.EquallySpacedRectSide\",\"uuid\":\"2833ed9d-c0e8-49c1-ad7b-8d4bc87d1df9\"},{\"content\":{\"connectorIds\":[],\"side\":\"HIDDEN\"},\"type\":\"ConnectorPlacement.EquallySpacedRectSide\",\"uuid\":\"76338804-e613-4140-a6be-ae9642a12407\"}]},\"type\":\"ConnectorPlacement.EquallySpacedConnector\",\"uuid\":\"276130fc-4c62-4f99-ae12-f3121ff878f4\"}],\"packageUris\":[\"http://schema.mathworks.com/mf0/Connector/R2020b\"],\"version\":\"1.0\"}"
      mask Display:
      | % Battery icon
      | plot([0 0 0.8 0.8], [0.2 0.9 0.9 1.5])
      | plot([0 0 0.8 0.8], -[0.2 0.9 0.9 1.5])
      | patch([-0.4 0.4 0.4 -0.4], [-0.45 -0.45 -0.15 -0.15], [0 0 0])
      | patch([-0.9 0.9 0.9 -0.9], [0.15 0.15 0.45 0.45], [0 0 0])
      | 
      | % Plot points to set plot range
      | color('white')
      | plot(1.5,1.5)
      | plot(-1.5,-1.5)
      | 
      | % Port labels
      | color('red')
      | port_label('LConn',1,'P')
      | port_label('LConn',2,'+')
      | port_label('RConn',1,'T')
      | port_label('RConn',2,'-')
  N : fl_lib/Physical Signals/Functions/PS Gain  gain=Ncells
  N-1 : fl_lib/Physical Signals/Functions/PS Gain  gain=Ncells - 1
  Thermal Model : Subsystem
  Voltage Sensor : fl_lib/Electrical/Electrical Sensors/Voltage Sensor
  - : PMIOPort  Side=Right
  H : PMIOPort  Port=2  Side=Left
  + : PMIOPort  Port=3  Side=Left
  connections:
  Lithium Cell 1RC/LConn1 -- N/LConn1
  Lithium Cell 1RC/RConn1 -- Thermal Model/RConn1
  Controlled Voltage Source/LConn1 -- Voltage Sensor/RConn2 -- Lithium Cell 1RC/RConn2
  Voltage Sensor/RConn1 -- N-1/LConn1
  Voltage Sensor/LConn1 -- Lithium Cell 1RC/LConn2 -- +/RConn1
  N-1/RConn1 -- Controlled Voltage Source/RConn1
  -/RConn1 -- Controlled Voltage Source/RConn2
  H/RConn1 -- Thermal Model/LConn1
  N/RConn1 -- Thermal Model/LConn2

== system ElectricVehicleThermalManagementWithHeatPump/Battery/Pack 4 ==
  note: Scale up voltage drop
      | to total of N cells
  Controlled Voltage Source : fl_lib/Electrical/Electrical Sources/Controlled Voltage Source
  Lithium Cell 1RC : Subsystem
      settings: PortSchema="{\"entries\":[{\"content\":{\"sides\":[{\"content\":{\"connectorIds\":[]},\"type\":\"ConnectorPlacement.EquallySpacedRectSide\",\"uuid\":\"ccb9f794-c2a7-49a2-9836-26607ca18a9f\"},{\"content\":{\"connectorIds\":[],\"side\":\"RIGHT\"},\"type\":\"ConnectorPlacement.EquallySpacedRectSide\",\"uuid\":\"f1620ab9-2b03-42d4-871e-d35b8093f316\"},{\"content\":{\"connectorIds\":[\"LConn1\",\"LConn2\"],\"side\":\"TOP\"},\"type\":\"ConnectorPlacement.EquallySpacedRectSide\",\"uuid\":\"e679b0d8-ccbe-4539-8d6b-f3ffcd05b92b\"},{\"content\":{\"connectorIds\":[\"RConn1\",\"RConn2\"],\"side\":\"BOTTOM\"},\"type\":\"ConnectorPlacement.EquallySpacedRectSide\",\"uuid\":\"2833ed9d-c0e8-49c1-ad7b-8d4bc87d1df9\"},{\"content\":{\"connectorIds\":[],\"side\":\"HIDDEN\"},\"type\":\"ConnectorPlacement.EquallySpacedRectSide\",\"uuid\":\"76338804-e613-4140-a6be-ae9642a12407\"}]},\"type\":\"ConnectorPlacement.EquallySpacedConnector\",\"uuid\":\"276130fc-4c62-4f99-ae12-f3121ff878f4\"}],\"packageUris\":[\"http://schema.mathworks.com/mf0/Connector/R2020b\"],\"version\":\"1.0\"}"
      mask Display:
      | % Battery icon
      | plot([0 0 0.8 0.8], [0.2 0.9 0.9 1.5])
      | plot([0 0 0.8 0.8], -[0.2 0.9 0.9 1.5])
      | patch([-0.4 0.4 0.4 -0.4], [-0.45 -0.45 -0.15 -0.15], [0 0 0])
      | patch([-0.9 0.9 0.9 -0.9], [0.15 0.15 0.45 0.45], [0 0 0])
      | 
      | % Plot points to set plot range
      | color('white')
      | plot(1.5,1.5)
      | plot(-1.5,-1.5)
      | 
      | % Port labels
      | color('red')
      | port_label('LConn',1,'P')
      | port_label('LConn',2,'+')
      | port_label('RConn',1,'T')
      | port_label('RConn',2,'-')
  N : fl_lib/Physical Signals/Functions/PS Gain  gain=Ncells
  N-1 : fl_lib/Physical Signals/Functions/PS Gain  gain=Ncells - 1
  Thermal Model : Subsystem
  Voltage Sensor : fl_lib/Electrical/Electrical Sensors/Voltage Sensor
  - : PMIOPort  Side=Right
  H : PMIOPort  Port=2  Side=Left
  + : PMIOPort  Port=3  Side=Left
  connections:
  N/RConn1 -- Thermal Model/LConn2
  H/RConn1 -- Thermal Model/LConn1
  -/RConn1 -- Controlled Voltage Source/RConn2
  N-1/RConn1 -- Controlled Voltage Source/RConn1
  +/RConn1 -- Lithium Cell 1RC/LConn2 -- Voltage Sensor/LConn1
  Voltage Sensor/RConn1 -- N-1/LConn1
  Lithium Cell 1RC/RConn2 -- Voltage Sensor/RConn2 -- Controlled Voltage Source/LConn1
  Lithium Cell 1RC/RConn1 -- Thermal Model/RConn1
  Lithium Cell 1RC/LConn1 -- N/LConn1

== system ElectricVehicleThermalManagementWithHeatPump/Battery/SB1 ==
  Heat Flow Rate Sensor : fl_lib/Thermal/Thermal Sensors/Heat Flow Rate Sensor
  PS-Simulink Converter : nesl_utility/PS-Simulink Converter  PhysicalDomain=network_engine_domain  SubClassName=ps_output  LeftPortType=input  RightPortType=output  PseudoPeriodic=off  Frequencies=[]  VectorFormat=inherit  Unit=degC  AffineConversion=on
  Temperature Sensor : fl_lib/Thermal/Thermal Sensors/Temperature Sensor  temperature_measure=foundation.enum.MeasurementReference.absolute
      settings: InternalSimscapePortConfiguration="{\"Bottom\":[],\"Left\":[{\"id\":\"A\",\"label\":\"A\",\"type\":\"foundation.thermal.thermal\"}],\"Right\":[{\"id\":\"T\",\"label\":\"T\",\"type\":\"output\"}],\"Top\":[]}"
  A : PMIOPort  Side=Left
  B : PMIOPort  Port=2  Side=Right
  tag scope: T_battery1=global
  wires:
  PS-Simulink Converter/1 -> [T_battery1]
  connections:
  A/RConn1 -- Heat Flow Rate Sensor/LConn1 -- Temperature Sensor/LConn1
  Heat Flow Rate Sensor/RConn2 -- B/RConn1
  PS-Simulink Converter/LConn1 -- Temperature Sensor/RConn1

== system ElectricVehicleThermalManagementWithHeatPump/Battery/SB2 ==
  Heat Flow Rate Sensor : fl_lib/Thermal/Thermal Sensors/Heat Flow Rate Sensor
  PS-Simulink Converter : nesl_utility/PS-Simulink Converter  PhysicalDomain=network_engine_domain  SubClassName=ps_output  LeftPortType=input  RightPortType=output  PseudoPeriodic=off  Frequencies=[]  VectorFormat=inherit  Unit=degC  AffineConversion=on
  Temperature Sensor : fl_lib/Thermal/Thermal Sensors/Temperature Sensor  temperature_measure=foundation.enum.MeasurementReference.absolute
      settings: InternalSimscapePortConfiguration="{\"Bottom\":[],\"Left\":[{\"id\":\"A\",\"label\":\"A\",\"type\":\"foundation.thermal.thermal\"}],\"Right\":[{\"id\":\"T\",\"label\":\"T\",\"type\":\"output\"}],\"Top\":[]}"
  A : PMIOPort  Side=Left
  B : PMIOPort  Port=2  Side=Right
  tag scope: T_battery2=global
  wires:
  PS-Simulink Converter/1 -> [T_battery2]
  connections:
  A/RConn1 -- Heat Flow Rate Sensor/LConn1 -- Temperature Sensor/LConn1
  Heat Flow Rate Sensor/RConn2 -- B/RConn1
  PS-Simulink Converter/LConn1 -- Temperature Sensor/RConn1

== system ElectricVehicleThermalManagementWithHeatPump/Battery/SB3 ==
  Heat Flow Rate Sensor : fl_lib/Thermal/Thermal Sensors/Heat Flow Rate Sensor
  PS-Simulink Converter : nesl_utility/PS-Simulink Converter  PhysicalDomain=network_engine_domain  SubClassName=ps_output  LeftPortType=input  RightPortType=output  PseudoPeriodic=off  Frequencies=[]  VectorFormat=inherit  Unit=degC  AffineConversion=on
  Temperature Sensor : fl_lib/Thermal/Thermal Sensors/Temperature Sensor  temperature_measure=foundation.enum.MeasurementReference.absolute
      settings: InternalSimscapePortConfiguration="{\"Bottom\":[],\"Left\":[{\"id\":\"A\",\"label\":\"A\",\"type\":\"foundation.thermal.thermal\"}],\"Right\":[{\"id\":\"T\",\"label\":\"T\",\"type\":\"output\"}],\"Top\":[]}"
  A : PMIOPort  Side=Left
  B : PMIOPort  Port=2  Side=Right
  tag scope: T_battery3=global
  wires:
  PS-Simulink Converter/1 -> [T_battery3]
  connections:
  A/RConn1 -- Heat Flow Rate Sensor/LConn1 -- Temperature Sensor/LConn1
  Heat Flow Rate Sensor/RConn2 -- B/RConn1
  PS-Simulink Converter/LConn1 -- Temperature Sensor/RConn1

== system ElectricVehicleThermalManagementWithHeatPump/Battery/SB4 ==
  Heat Flow Rate Sensor : fl_lib/Thermal/Thermal Sensors/Heat Flow Rate Sensor
  PS-Simulink Converter : nesl_utility/PS-Simulink Converter  PhysicalDomain=network_engine_domain  SubClassName=ps_output  LeftPortType=input  RightPortType=output  PseudoPeriodic=off  Frequencies=[]  VectorFormat=inherit  Unit=degC  AffineConversion=on
  Temperature Sensor : fl_lib/Thermal/Thermal Sensors/Temperature Sensor  temperature_measure=foundation.enum.MeasurementReference.absolute
      settings: InternalSimscapePortConfiguration="{\"Bottom\":[],\"Left\":[{\"id\":\"A\",\"label\":\"A\",\"type\":\"foundation.thermal.thermal\"}],\"Right\":[{\"id\":\"T\",\"label\":\"T\",\"type\":\"output\"}],\"Top\":[]}"
  A : PMIOPort  Side=Left
  B : PMIOPort  Port=2  Side=Right
  tag scope: T_battery4=global
  wires:
  PS-Simulink Converter/1 -> [T_battery4]
  connections:
  A/RConn1 -- Heat Flow Rate Sensor/LConn1 -- Temperature Sensor/LConn1
  Heat Flow Rate Sensor/RConn2 -- B/RConn1
  PS-Simulink Converter/LConn1 -- Temperature Sensor/RConn1

== system ElectricVehicleThermalManagementWithHeatPump/Battery/SC3 ==
  Flow Rate Sensor (TL) : fl_lib/Thermal Liquid/Sensors/Flow Rate Sensor (TL)  mass_flow_measure=true  volumetric_flow_measure=false  energy_flow_measure=true
      settings: InternalSimscapePortConfiguration="{\"Bottom\":[{\"id\":\"PHI\",\"label\":\"φ\",\"type\":\"output\"}],\"Left\":[{\"id\":\"A\",\"label\":\"A\",\"type\":\"foundation.thermal_liquid.thermal_liquid\"}],\"Right\":[{\"id\":\"B\",\"label\":\"B\",\"type\":\"foundation.thermal_liquid.thermal_liquid\"},{\"id\":\"M\",\"label\":\"M\",\"type\":\"output\"}],\"Top\":[]}"
  PS-Simulink Converter : nesl_utility/PS-Simulink Converter  PhysicalDomain=network_engine_domain  SubClassName=ps_output  LeftPortType=input  RightPortType=output  PseudoPeriodic=off  Frequencies=[]  VectorFormat=inherit  Unit=W  AffineConversion=off
  PS-Simulink Converter1 : nesl_utility/PS-Simulink Converter  PhysicalDomain=network_engine_domain  SubClassName=ps_output  LeftPortType=input  RightPortType=output  PseudoPeriodic=off  Frequencies=[]  VectorFormat=inherit  Unit=degC  AffineConversion=on
  PS-Simulink Converter2 : nesl_utility/PS-Simulink Converter  PhysicalDomain=network_engine_domain  SubClassName=ps_output  LeftPortType=input  RightPortType=output  PseudoPeriodic=off  Frequencies=[]  VectorFormat=inherit  Unit=inherit  AffineConversion=off
  Pressure & Temperature Sensor (TL) : fl_lib/Thermal Liquid/Sensors/Pressure & Temperature Sensor (TL)  reference=foundation.enum.MeasurementReference.absolute  pressure=true  pressure_spec=foundation.enum.PressureMeasementSpec.Absolute  temperature=true
      settings: InternalSimscapePortConfiguration="{\"Bottom\":[{\"id\":\"T\",\"label\":\"T\",\"type\":\"output\"}],\"Left\":[{\"id\":\"A\",\"label\":\"A\",\"type\":\"foundation.thermal_liquid.thermal_liquid\"}],\"Right\":[{\"id\":\"Pa\",\"label\":\"Pa\",\"type\":\"output\"}],\"Top\":[]}"
  Scope : Scope
  A : PMIOPort  Side=Left
  B : PMIOPort  Port=2  Side=Right
  tag scope: Phi_battery_in=global, T_coolant_battery_in=global
  wires:
  PS-Simulink Converter/1 -> [Phi_battery_in]
  PS-Simulink Converter1/1 -> [T_coolant_battery_in]
  PS-Simulink Converter2/1 -> Scope/1
  connections:
  PS-Simulink Converter/LConn1 -- Flow Rate Sensor (TL)/RConn3
  A/RConn1 -- Pressure & Temperature Sensor (TL)/LConn1 -- Flow Rate Sensor (TL)/LConn1
  B/RConn1 -- Flow Rate Sensor (TL)/RConn1
  PS-Simulink Converter1/LConn1 -- Pressure & Temperature Sensor (TL)/RConn2
  PS-Simulink Converter2/LConn1 -- Flow Rate Sensor (TL)/RConn2

== system ElectricVehicleThermalManagementWithHeatPump/Battery/SC4 ==
  Flow Rate Sensor (TL) : fl_lib/Thermal Liquid/Sensors/Flow Rate Sensor (TL)  mass_flow_measure=true  volumetric_flow_measure=false  energy_flow_measure=true
      settings: InternalSimscapePortConfiguration="{\"Bottom\":[{\"id\":\"PHI\",\"label\":\"φ\",\"type\":\"output\"}],\"Left\":[{\"id\":\"A\",\"label\":\"A\",\"type\":\"foundation.thermal_liquid.thermal_liquid\"}],\"Right\":[{\"id\":\"B\",\"label\":\"B\",\"type\":\"foundation.thermal_liquid.thermal_liquid\"},{\"id\":\"M\",\"label\":\"M\",\"type\":\"output\"}],\"Top\":[]}"
  PS-Simulink Converter : nesl_utility/PS-Simulink Converter  PhysicalDomain=network_engine_domain  SubClassName=ps_output  LeftPortType=input  RightPortType=output  PseudoPeriodic=off  Frequencies=[]  VectorFormat=inherit  Unit=W  AffineConversion=off
  Pressure & Temperature Sensor (TL) : fl_lib/Thermal Liquid/Sensors/Pressure & Temperature Sensor (TL)  reference=foundation.enum.MeasurementReference.absolute  pressure=true  pressure_spec=foundation.enum.PressureMeasementSpec.Absolute  temperature=true
      settings: InternalSimscapePortConfiguration="{\"Bottom\":[{\"id\":\"T\",\"label\":\"T\",\"type\":\"output\"}],\"Left\":[{\"id\":\"A\",\"label\":\"A\",\"type\":\"foundation.thermal_liquid.thermal_liquid\"}],\"Right\":[{\"id\":\"Pa\",\"label\":\"Pa\",\"type\":\"output\"}],\"Top\":[]}"
  A : PMIOPort  Side=Left
  B : PMIOPort  Port=2  Side=Right
  tag scope: Phi_battery_out=global
  wires:
  PS-Simulink Converter/1 -> [Phi_battery_out]
  connections:
  B/RConn1 -- Flow Rate Sensor (TL)/RConn1
  Flow Rate Sensor (TL)/LConn1 -- Pressure & Temperature Sensor (TL)/LConn1 -- A/RConn1
  PS-Simulink Converter/LConn1 -- Flow Rate Sensor (TL)/RConn3
